simulink model "physical_lab5_frequency_second"  (R2024b)
settings: Solver=ode15s  StartTime=0.0  StopTime=2.8571428571428572  MaxStep=0.00047619047619047619  RelTol=1e-7  AbsTol=1e-9
model workspace (MAT data in the model file):
  physical_input = timeseries
  physical_input.Name = 'unnamed'
  physical_input.DataInfo = tsdata.datametadata
  physical_input.DataInfo.Interpolation = tsdata.interpolation
  physical_input.DataInfo.Interpolation.Fhandle : function handle (value not decoded)
  physical_input.DataInfo.Interpolation.Name = 'linear'
  physical_input.TimeInfo = tsdata.timemetadata
  physical_input.TimeInfo.Length = 6001
  physical_input.TimeInfo.DuplicateTimes = 0
  physical_input.TimeInfo.Time_ = [0 0.00047619047619 0.000952380952381 0.00142857142857 0.00190476190476 0.00238095238095 0.00285714285714 0.00333333333333 0.00380952380952 0.00428571428571 0.0047619047619 0.0052380952381 ... (6001 elements, 6001x1)]
  physical_input.TimeInfo.Initialized = 1
  physical_input.QualityInfo = tsdata.qualmetadata
  physical_input.Data_ = [0 0.0104717841162 0.0209424198834 0.0314107590781 0.0418756537292 0.0523359562429 0.0627905195293 0.0732381971276 0.0836778433323 0.0941083133185 0.104528463268 0.114937150493 ... (6001 elements, 6001x1)]
libraries: fl_lib x17, nesl_utility x3
settings Model: Creator=33657  LastModifiedBy=33657

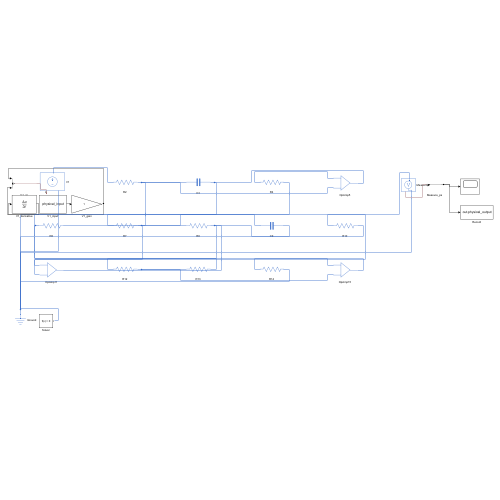
[thumbnail: Simulink's stored preview of the top-level diagram]
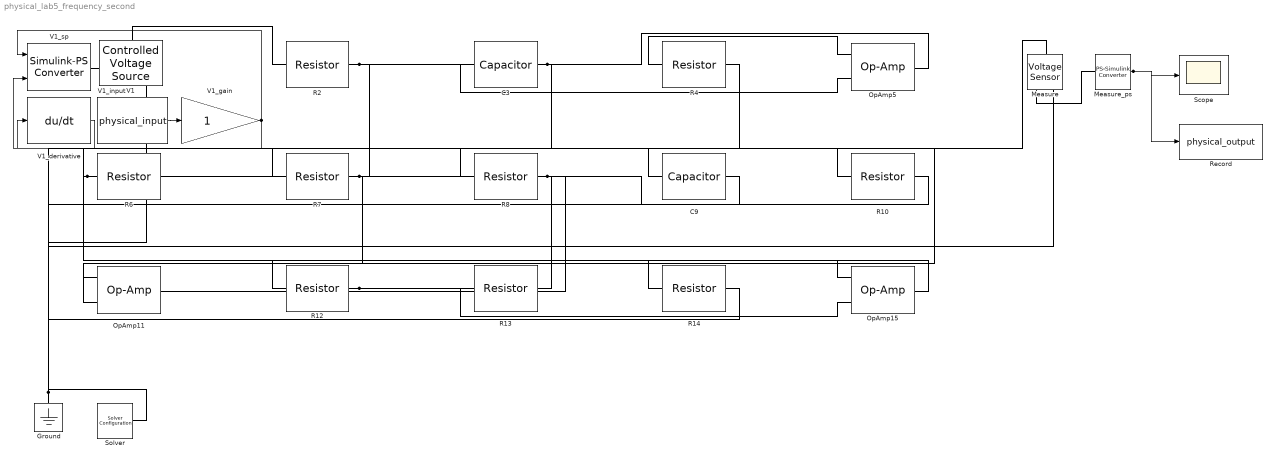
== system physical_lab5_frequency_second ==
  C3 : fl_lib/Electrical/Electrical Elements/Capacitor  c=9.9999999999999995e-07 F  r=0 Ohm  g=0 1/Ohm  i_specify=off  i_priority=None  i=0 A  i_nominal_specify=off  i_nominal_value=1  i_nominal_unit=A  v_specify=off  v_priority=None  v=0 V  v_nominal_specify=off  v_nominal_value=1  v_nominal_unit=V  vc_specify=off  vc_priority=High  vc=0 V  vc_nominal_specify=off  vc_nominal_value=1  vc_nominal_unit=V
  C9 : fl_lib/Electrical/Electrical Elements/Capacitor  c=9.9999999999999995e-07 F  r=0 Ohm  g=0 1/Ohm  i_specify=off  i_priority=None  i=0 A  i_nominal_specify=off  i_nominal_value=1  i_nominal_unit=A  v_specify=off  v_priority=None  v=0 V  v_nominal_specify=off  v_nominal_value=1  v_nominal_unit=V  vc_specify=off  vc_priority=High  vc=0 V  vc_nominal_specify=off  vc_nominal_value=1  vc_nominal_unit=V
  Ground : fl_lib/Electrical/Electrical Elements/Electrical Reference
  Measure : fl_lib/Electrical/Electrical Sensors/Voltage Sensor
  Measure_ps : nesl_utility/PS-Simulink Converter  PhysicalDomain=network_engine_domain  SubClassName=ps_output  LeftPortType=input  RightPortType=output  PseudoPeriodic=off  Frequencies=[]  VectorFormat=inherit  Unit=V  AffineConversion=off
  OpAmp11 : fl_lib/Electrical/Electrical Elements/Op-Amp  outI_specify=off  outI_priority=None  outI=0 A  outI_nominal_specify=off  outI_nominal_value=1  outI_nominal_unit=A
  OpAmp15 : fl_lib/Electrical/Electrical Elements/Op-Amp  outI_specify=off  outI_priority=None  outI=0 A  outI_nominal_specify=off  outI_nominal_value=1  outI_nominal_unit=A
  OpAmp5 : fl_lib/Electrical/Electrical Elements/Op-Amp  outI_specify=off  outI_priority=None  outI=0 A  outI_nominal_specify=off  outI_nominal_value=1  outI_nominal_unit=A
  R{2,4,6..8,10,12,14} (8 alike) : fl_lib/Electrical/Electrical Elements/Resistor  R=100000 Ohm  i_specify=off  i_priority=None  i=0 A  i_nominal_specify=off  i_nominal_value=1  i_nominal_unit=A  v_specify=off  v_priority=None  v=0 V  v_nominal_specify=off  v_nominal_value=1  v_nominal_unit=V
  R13 : fl_lib/Electrical/Electrical Elements/Resistor  R=500000.00000000006 Ohm  i_specify=off  i_priority=None  i=0 A  i_nominal_specify=off  i_nominal_value=1  i_nominal_unit=A  v_specify=off  v_priority=None  v=0 V  v_nominal_specify=off  v_nominal_value=1  v_nominal_unit=V
  Record : ToWorkspace  VariableName=physical_output  SaveFormat=Timeseries  SampleTime=-1
  Scope : Scope
  Solver : nesl_utility/Solver Configuration  PhysicalDomain=network_engine_domain  SubClassName=solver  LeftPortType=input  RightPortType=generic  Tones=[]  Harmonics=[]  SimulateNoise=off  Profile=off  UseLocalSampling=off  EnableSwitchedLinearOptims=on  FrequencyDomain=off  UseCCode=off  RelTol=0.001  AbsTol=0.001  MinStep=1e-09  ToWorkspace=off  RevertToSquareIcSolve=off  NumHomotopyIterations=100  PhasorMode=off  PhasorModeNumHarmonics=1  ConsistencySolver=NEWTON_XTOL_AFTER_FTOL  IndexReductionMethod=DerivativeReplacement  DoDC=off  ResidualTolerance=1e-09  ConsistencyTolSource=GLOBAL  ConsistencyAbsTol=0.001  ConsistencyRelTol=0.001  ConsistencyTolFactor=0.001  UseLocalSolver=off  LocalSolverChoice=NE_BACKWARD_EULER_ADVANCER  ResolveIndetEquations=on  FunctionEvalNumThread=1  LocalSolverSampleTime=0.001  DoFixedCost=off  MaxNonlinIter=3  MaxModeIter=2  ComputeImpulses=off  ImpulseIterations=2  LinearAlgebra=auto  LinearAlgebraNumThread=0  EquationFormulation=NE_TIME_EF  DelaysMemoryBudget=1024  AutomaticFiltering=on  FilteringTimeConstant=0.001  PartitionStorageMethod=AS_NEEDED  PartitionMemoryBudget=1024  PartitionMethod=ROBUST  MultibodyUseLocalSolver=off  MultibodyLocalSolverChoice=ODE1  MultibodyLocalSolverSampleTime=0.001
  V1 : fl_lib/Electrical/Electrical Sources/Controlled Voltage Source
  V1_derivative : Derivative
  V1_gain : Gain
  V1_input : FromWorkspace  VariableName=physical_input
  V1_sp : nesl_utility/Simulink-PS Converter  PhysicalDomain=network_engine_domain  SubClassName=ps_input  LeftPortType=input  RightPortType=output  PseudoPeriodic=off  Frequencies=[]  NoiseDistribution=none  NoiseParameters=[]  Unit=V  AffineConversion=off  FilteringAndDerivatives=provide  SimscapeFilterOrder=1  InputFilterTimeConstant=0.001  UdotUserProvided=1
  wires:
  V1_input/1 -> V1_gain/1
  V1_gain/1 -> V1_derivative/1, V1_sp/1
  V1_derivative/1 -> V1_sp/2
  Measure_ps/1 -> Scope/1, Record/1
  connections:
  Solver/RConn1 -- Ground/LConn1 -- V1/RConn2 -- R4/RConn1 -- R10/RConn1 -- R14/RConn1 -- Measure/RConn2
  V1_sp/RConn1 -- V1/RConn1
  V1/LConn1 -- R2/LConn1
  C3/LConn1 -- R2/RConn1 -- OpAmp5/LConn2 -- R6/RConn1
  R4/LConn1 -- OpAmp5/LConn1
  OpAmp5/RConn1 -- C3/RConn1 -- R7/LConn1
  R8/LConn1 -- R7/RConn1 -- C9/LConn1 -- OpAmp11/LConn2
  C9/RConn1 -- R8/RConn1 -- OpAmp11/RConn1 -- R12/LConn1
  R10/LConn1 -- OpAmp11/LConn1
  R13/LConn1 -- R12/RConn1 -- OpAmp15/LConn2
  R13/RConn1 -- R6/LConn1 -- OpAmp15/RConn1 -- Measure/LConn1
  R14/LConn1 -- OpAmp15/LConn1
  Measure/RConn1 -- Measure_ps/LConn1
